simulink model "EMT"  (R2024b)
settings: Solver=ode5  StartTime=0.0  StopTime=1500  FixedStep=0.002  RelTol=1e-3
PreLoadFcn:
  | parameter;
InitFcn:
  | parameter;
StopFcn:
  | save('result.mat');
values from neighbouring files (symbols this model uses):
  A = 7.3    [parameter.m]
  a11 = (1+k1)*(1+k2)/k1/k2/iq    (= 1.54241568346)    [parameter.m]
  a11_L = a11    (= 1.54241568346)    [parameter.m]
  a12 = -(1+k1+k2)*(1+k3)/k1/k2    (= -3.86074191629)    [parameter.m]
  a12_L = a11*(1+k3+k4)/(1+k3)    (= 2.43173643789)    [parameter.m]
  a21 = -(1+k2)/k1/iq    (= -1.04963112005)    [parameter.m]
  a22 = (1+k1+k2)/k1    (= 2.46948356808)    [parameter.m]
  B = 2.71    [parameter.m]
  b11 = 0    [parameter.m]
  b12 = (1+k3)    (= 3.33)    [parameter.m]
  b21 = (1+k2)/iq    (= 2.23571428571)    [parameter.m]
  b22 = -k2    (= -2.13)    [parameter.m]
  C1_shift = 200    [parameter.m]
  Cb = 70    [parameter.m]
  Cd = 0.6    [parameter.m]
  eff_generator = eff_motor    [parameter.m]
  eff_motor = [0.80 0.80 0.84 0.84 0.83 0.85 0.83 0.83 0.83 0.80 0.80 0.80 ... (first row only)    [parameter.m]
  ele_map = [10.00,11.46,14.13,19.24,20.94,23.21,20.29,20.23,22.28,17.66,16.24,18.95,20.79,16.98,18.22,16.52,18.29,20.67,20.82,23.14,23.36,21.30,17.71,20.26,19.53,21.18,23.13,22.79,19.35,16.77,20.50,19.02,20.56,21.90,23.91,20.40,18.45,22.70,22.38,22.48,21.84,17.76,20.13,22.61,19.35,19.36,21.56,20.37,18.38,17.96,18.38,17.24,18.99,22.31,23.50,18.24,22.11,20.73,20.35,18.91,22.88,20.92,18.75,16.85,21.94,17.80,19. ...(+2007 chars)    [parameter.m]
  Fb_max = 5.5*mass    (= 247500)    [parameter.m]
  ic = 4.42    [parameter.m]
  JA = 0.4    [parameter.m]
  JB = JA    (= 0.4)    [parameter.m]
  Jc3r4 = 1e-2    (= 0.01)    [parameter.m]
  Je = 2.5    [parameter.m]
  Jh = 1e-2    (= 0.01)    [parameter.m]
  kh = 2.88    [parameter.m]
  kt = 1.83    [parameter.m]
  L = 4.472    [parameter.m]
  mass = 45000    [parameter.m]
  miu_max = 0.8    [parameter.m]
  n_generator = n_motor    [parameter.m]
  n_motor = [0 0.1 0.25 0.4 0.55 0.7 0.85 1 1.15 1.3 1.45 2.2]*3185    [parameter.m]
  nA_map = [-6000:50:-3250 -3200 0 3200 3250:50:6000]    [parameter.m]    (also in plot_result.m = [-7000:50:-3250 -3200 0 3200 3250:50:7000])
  nA_max = max(nA_map)    [parameter.m]
  nA_min = min(nA_map)    [parameter.m]
  nB_map = nA_map    [parameter.m]    (also in plot_result.m = [-7000:50:-3250 -3200 0 3200 3250:50:7000])
  nB_max = nA_max    [parameter.m]
  nB_min = nA_min    [parameter.m]
  ne_idl = 3000    [parameter.m]
  ne_map = [1600,1700,1800,1900,2000,2100,2200,2300,2400,2500,2600,2700,2800,2900,3000,3100,3200,3300,3400,3500,3600,3700,3800,3900,4000,4100,4200,4500]    [parameter.m]
  ne_max = 4200    [parameter.m]
  ne_min = 1600    [parameter.m]
  ne_start = 200    [parameter.m]
  nZ_map = [-8000:50:-4850 -4800 0 4800 4850:50:8000]    [parameter.m]
  Pb_epr = [-45 -45 -40 -30 0 30 40 45 45]    [parameter.m]
  Pb_max = [0 40 45 45 45]    [parameter.m]
  Pb_min = [-45 -45 -45 -40 0]    [parameter.m]
  Pe_ass = 210+20    (= 230)    [parameter.m]
  Pe_max = 1103    [parameter.m]
  PN0 = 0    [parameter.m]
  R_map = [0.90 0.89 0.90 0.91 0.92 0.93 0.94 0.95 0.96 0.97 0.98]/10    [parameter.m]
  rz = 0.318    [parameter.m]
  SOC0 = 60    [parameter.m]
  SOC_epr = [30 31 50 59 60 61 70 79 80]    [parameter.m]
  SOC_map = 0:10:100    [parameter.m]
  T_generator = T_motor    [parameter.m]
  T_motor = [0 0.3 0.8 1.3 1.8 2.3 2.8]/1.8*1110    [parameter.m]
  TA_max_map = [370*9549./(6000:-50:3250) 1110 1110 1110 370*9549./(3250:50:6000)]    [parameter.m]    (also in plot_result.m = [370*9549./(7000:-50:3250) 1100 1100 1100 370*9549./(3250:50)
  TA_min_map = -TA_max_map    [parameter.m]
  TAf = 0    [parameter.m]
  TB_max_map = TA_max_map    [parameter.m]    (also in plot_result.m = [370*9549./(7000:-50:3250) 1110 1110 1110 370*9549./(3250:50)
  TB_min_map = TA_min_map    [parameter.m]
  TBf = TAf    (= 0)    [parameter.m]
  Te_map = [0,599,798,998,1168,1324,1495,1660,1822,1970,2106,2235,2355,2458,2508,2543,2565,2606,2613,2649,2658,2689,2701,2707,2719,2724,2728,2740,2743,2754]    [parameter.m]
  Te_max_map = [1168,1324,1495,1660,1822,1970,2106,2235,2355,2458,2543,2606,2658,2701,2728,2743,2754,2743,2740,2724,2719,2707,2689,2649,2613,2565,2508,998]    [parameter.m]
  Te_start = 1600    [parameter.m]
  Tef = 100    [parameter.m]
  Time = 0:0.1:200    [parameter.m]
  Time_ele = 0:4:1600    [parameter.m]
  TS_A = 0.2    [parameter.m]
  TS_B = TS_A    (= 0.2)    [parameter.m]
  TS_C0 = 0.2    [parameter.m]
  TS_C1 = 0.2    [parameter.m]
  Ts_e = 0.1    [parameter.m]
  TS_Z1 = 0.2    [parameter.m]
  TS_Z2 = 0.2    [parameter.m]
  TZ_max_map = [450*9549./(8000:-50:4850) 1000 1000 1000 450*9549./(4850:50:8000)]    [parameter.m]
  TZ_min_map = -TZ_max_map    [parameter.m]
  Uoc_map = [3.258,3.668,3.733,3.783,3.833,3.877,3.912,3.941,3.973,4.013,4.200]*250    [parameter.m]
  v_cyc = 0.*(0<=Time&Time<11)+(3.75.*Time-41.25).*(11<=Time&Time<15)+15.*(15<=Time&Time<23)+(-3.*Time+84).*(23<=Time&Time<28)+0.*(28<=Time&Time<49)+(8.*Time/3-392/3).*(49<=Time&Time<61)+32.*(61<=Time&Time<85)+(-32.*Time/11+3072/11).*(85<=Time&Time<96)+0.*(96<=Time&Time<117)+(25.*Time/13-2925/13).*(117<=Time&Time<143)+50.*(143<=Time&Time<155)+(-15.*Time/8+2725/8).*(155<=Time&Time<163)+35.*(163<=Time&Time<17 ...(+70 chars)    [parameter.m]
  V_Shift12 = 32    [parameter.m]
  V_Shift21 = 25    [parameter.m]
  Voltage_epr = [750 760 900 1000 1050]    [parameter.m]
  Y_engine = 0.955    [parameter.m]
  Yc = 0.98    [parameter.m]
  Yh = 0.96    [parameter.m]
  Z1_shift = 200    [parameter.m]
  Z2_shift = 200    [parameter.m]
undefined symbols (not defined in the file or in its folder): sigbuilder_block
libraries: fl_lib x82, nesl_utility x55, simulink x49, sdl_lib x10, simulink_need_slupdate x6, powerlib_extras x1
(part 4 of 6)

== system EMT/Vehicle dynamics/vehicle dynamic/vehicle dynamic/Torque Actuator ==
  torque : Inport
  Ideal Torque Source : fl_lib/Mechanical/Mechanical Sources/Ideal Torque Source
  Mechanical Rotational Reference : fl_lib/Mechanical/Rotational Elements/Mechanical Rotational Reference
  Simulink-PS Converter : nesl_utility/Simulink-PS Converter  PhysicalDomain=network_engine_domain  SubClassName=ps_input  LeftPortType=input  RightPortType=output  PseudoPeriodic=off  Frequencies=[]  NoiseDistribution=none  NoiseParameters=[]  Unit=1  AffineConversion=off  FilteringAndDerivatives=filter  SimscapeFilterOrder=2  InputFilterTimeConstant=.001  UdotUserProvided=1
  shaft : PMIOPort  Side=Right
  wires:
  torque/1 -> Simulink-PS Converter/1
  connections:
  Simulink-PS Converter/RConn1 -- Ideal Torque Source/RConn1
  Mechanical Rotational Reference/LConn1 -- Ideal Torque Source/RConn2
  shaft/RConn1 -- Ideal Torque Source/LConn1

== system EMT/Vehicle dynamics/vehicle dynamic/vehicle dynamic/Torque Sensor ==
  Ideal Torque Sensor : fl_lib/Mechanical/Mechanical Sensors/Ideal Torque Sensor
  PS-Simulink Converter : nesl_utility/PS-Simulink Converter  PhysicalDomain=network_engine_domain  SubClassName=ps_output  LeftPortType=input  RightPortType=output  PseudoPeriodic=off  Frequencies=[]  VectorFormat=1-D array  Unit=1  AffineConversion=off
  In : PMIOPort  Side=Left
  Out : PMIOPort  Port=2  Side=Right
  Nm : Outport
  wires:
  PS-Simulink Converter/1 -> Nm/1
  connections:
  PS-Simulink Converter/LConn1 -- Ideal Torque Sensor/RConn2
  In/RConn1 -- Ideal Torque Sensor/LConn1
  Ideal Torque Sensor/RConn1 -- Out/RConn1

== system EMT/Vehicle dynamics/vehicle dynamic/vehicle dynamic/Wind Resistance ==
  Air Resistance : Fcn  Expr=0.5*Cd*A*u*u/21.15
  Memory3 : Memory
  Fw : Outport
  wires:
  [v_act] -> Memory3/1
  Memory3/1 -> Air Resistance/1
  Air Resistance/1 -> Fw/1

== system EMT/Vehicle dynamics/vehicle dynamic/vehicle dynamic1/Grade Resistance ==
  angle : Inport
  Ground Resistance : Fcn  Expr=0.5*mass*9.8*sin(u)
  Fg : Outport
  wires:
  angle/1 -> Ground Resistance/1
  Ground Resistance/1 -> Fg/1

== system EMT/Vehicle dynamics/vehicle dynamic/vehicle dynamic1/Ground Resistance ==
  fg : Inport
  angle : Inport  Port=2
  Ground Resistance : Fcn  Expr=0.5*u(1)*mass*9.8*cos(u(2))
  Mux : Mux  Inputs=2
  Ff : Outport
  wires:
  angle/1 -> Mux/2
  fg/1 -> Mux/1
  Mux/1 -> Ground Resistance/1
  Ground Resistance/1 -> Ff/1

== system EMT/Vehicle dynamics/vehicle dynamic/vehicle dynamic1/Mode Judge ==
  v : Inport
  Add : Sum  Inputs=+++
  Compare To Constant1 : simulink/Logic and Bit Operations/Compare To Constant  relop=<  const=-0.1  OutDataTypeStr=uint8
  Compare To Constant2 : simulink/Logic and Bit Operations/Compare To Constant  relop=>  const=0.1  OutDataTypeStr=uint8
  Compare To Constant3 : simulink/Logic and Bit Operations/Compare To Constant  relop=>=  const=-0.1  OutDataTypeStr=uint8
  Compare To Constant4 : simulink/Logic and Bit Operations/Compare To Constant  relop=<=  const=0.1  OutDataTypeStr=uint8
  Data Type Conversion : DataTypeConversion  SaturateOnIntegerOverflow=off  RndMeth=Floor
  Gain : Gain  Gain=3
  Gain1 : Gain  Gain=2
  Gain2 : Gain
  Logical Operator : Logic  AllPortsSameDT=off  OutDataTypeStr=boolean
  F : Outport
  wires:
  Gain2/1 -> Add/1
  Gain/1 -> Add/3
  Data Type Conversion/1 -> F/1
  Logical Operator/1 -> Gain/1
  Compare To Constant2/1 -> Gain1/1
  Compare To Constant4/1 -> Logical Operator/2
  Compare To Constant3/1 -> Logical Operator/1
  Compare To Constant1/1 -> Gain2/1
  v/1 -> Compare To Constant1/1, Compare To Constant2/1, Compare To Constant3/1, Compare To Constant4/1
  Add/1 -> Data Type Conversion/1
  Gain1/1 -> Add/2

== system EMT/Vehicle dynamics/vehicle dynamic/vehicle dynamic1/Speed Sensor ==
  Ideal Rotational Motion Sensor : fl_lib/Mechanical/Mechanical Sensors/Ideal Rotational Motion Sensor  reference=foundation.enum.MeasurementReference.difference  acceleration_port=false  velocity_port=true  position_port=true  wrap_angle=false  offset=0 rad
  PS-Simulink Converter : nesl_utility/PS-Simulink Converter  PhysicalDomain=network_engine_domain  SubClassName=ps_output  LeftPortType=input  RightPortType=output  PseudoPeriodic=off  Frequencies=[]  VectorFormat=1-D array  Unit=1  AffineConversion=off
  Reference : fl_lib/Mechanical/Rotational Elements/Mechanical Rotational Reference
  Tire Radius2 : Gain  Gain=30/pi
  shaft : PMIOPort  Side=Left
  r/min : Outport
  wires:
  PS-Simulink Converter/1 -> Tire Radius2/1
  Tire Radius2/1 -> r/min/1
  connections:
  PS-Simulink Converter/LConn1 -- Ideal Rotational Motion Sensor/RConn2
  Reference/LConn1 -- Ideal Rotational Motion Sensor/RConn1
  shaft/RConn1 -- Ideal Rotational Motion Sensor/LConn1

== system EMT/Vehicle dynamics/vehicle dynamic/vehicle dynamic1/Steering Resistance ==
  Abs : Abs  SaturateOnIntegerOverflow=off
  Compare To Constant : simulink/Logic and Bit Operations/Compare To Constant  relop=>=  const=10^3  OutDataTypeStr=uint8  ZeroCross=off
  Constant1 : Constant  Value=0
  Memory1 : Memory
  Memory3 : Memory
  Mux : Mux  Inputs=2
  Product2 : Product  RndMeth=Zero
  Sign1 : Signum
  Steering Resistance : Fcn  Expr=miu_max/(0.925+0.15*(u))*mass*9.8*L/4/B
  Switch : Switch  Threshold=0.5  SaturateOnIntegerOverflow=off  InputSameDT=off
  rou : Fcn  Expr=(u(1)+u(2))/(u(2)-u(1)+0.1^10)/2
  Fs : Outport
  wires:
  [v_Right] -> Memory1/1
  [v_Left] -> Memory3/1
  Product2/1 -> Fs/1
  Sign1/1 -> Switch/3
  Switch/1 -> Product2/2
  Constant1/1 -> Switch/1
  Compare To Constant/1 -> Switch/2
  Abs/1 -> Steering Resistance/1  "rou"
  rou/1 -> Sign1/1, Compare To Constant/1, Abs/1
  Mux/1 -> rou/1
  Memory1/1 -> Mux/2
  Memory3/1 -> Mux/1
  Steering Resistance/1 -> Product2/1

== system EMT/Vehicle dynamics/vehicle dynamic/vehicle dynamic1/Torque Actuator ==
  torque : Inport
  Ideal Torque Source : fl_lib/Mechanical/Mechanical Sources/Ideal Torque Source
  Mechanical Rotational Reference : fl_lib/Mechanical/Rotational Elements/Mechanical Rotational Reference
  Simulink-PS Converter : nesl_utility/Simulink-PS Converter  PhysicalDomain=network_engine_domain  SubClassName=ps_input  LeftPortType=input  RightPortType=output  PseudoPeriodic=off  Frequencies=[]  NoiseDistribution=none  NoiseParameters=[]  Unit=1  AffineConversion=off  FilteringAndDerivatives=filter  SimscapeFilterOrder=2  InputFilterTimeConstant=.001  UdotUserProvided=1
  shaft : PMIOPort  Side=Right
  wires:
  torque/1 -> Simulink-PS Converter/1
  connections:
  shaft/RConn1 -- Ideal Torque Source/LConn1
  Mechanical Rotational Reference/LConn1 -- Ideal Torque Source/RConn2
  Simulink-PS Converter/RConn1 -- Ideal Torque Source/RConn1

== system EMT/Vehicle dynamics/vehicle dynamic/vehicle dynamic1/Torque Sensor ==
  Ideal Torque Sensor : fl_lib/Mechanical/Mechanical Sensors/Ideal Torque Sensor
  PS-Simulink Converter : nesl_utility/PS-Simulink Converter  PhysicalDomain=network_engine_domain  SubClassName=ps_output  LeftPortType=input  RightPortType=output  PseudoPeriodic=off  Frequencies=[]  VectorFormat=1-D array  Unit=1  AffineConversion=off
  In : PMIOPort  Side=Left
  Out : PMIOPort  Port=2  Side=Right
  Nm : Outport
  wires:
  PS-Simulink Converter/1 -> Nm/1
  connections:
  Ideal Torque Sensor/RConn1 -- Out/RConn1
  In/RConn1 -- Ideal Torque Sensor/LConn1
  PS-Simulink Converter/LConn1 -- Ideal Torque Sensor/RConn2

== system EMT/Vehicle dynamics/vehicle dynamic/vehicle dynamic1/Wind Resistance ==
  Air Resistance : Fcn  Expr=0.5*Cd*A*u*u/21.15
  Memory3 : Memory
  Fw : Outport
  wires:
  [v_act] -> Memory3/1
  Memory3/1 -> Air Resistance/1
  Air Resistance/1 -> Fw/1

== system EMT/engine/Engine/Subsystem1/Torque Actuator ==
  torque : Inport
  Ideal Torque Source : fl_lib/Mechanical/Mechanical Sources/Ideal Torque Source
  Mechanical Rotational Reference : fl_lib/Mechanical/Rotational Elements/Mechanical Rotational Reference
  Simulink-PS Converter : nesl_utility/Simulink-PS Converter  PhysicalDomain=network_engine_domain  SubClassName=ps_input  LeftPortType=input  RightPortType=output  PseudoPeriodic=off  Frequencies=[]  NoiseDistribution=none  NoiseParameters=[]  Unit=N*m  AffineConversion=off  FilteringAndDerivatives=zero  SimscapeFilterOrder=1  InputFilterTimeConstant=.001  UdotUserProvided=0
  shaft : PMIOPort  Side=Right
  wires:
  torque/1 -> Simulink-PS Converter/1
  connections:
  Simulink-PS Converter/RConn1 -- Ideal Torque Source/RConn1
  Mechanical Rotational Reference/LConn1 -- Ideal Torque Source/RConn2
  shaft/RConn1 -- Ideal Torque Source/LConn1

== system EMT/motorA/Motor/Mechanical Body/Max & Min Torque Control ==
  speed : Inport
  Tm_com : Inport  Port=2
  Lookup Table : Lookup  InputValues=nm_map  Table=Tm_max_map  SaturateOnIntegerOverflow=off
  Lookup Table1 : Lookup  InputValues=nm_map  Table=Tm_min_map  SaturateOnIntegerOverflow=off
  Saturation Dynamic : simulink/Discontinuities/Saturation Dynamic  OutMin=[]  OutMax=[]  OutDataTypeStr=Inherit: Same as second input  OutDataType=sfix(16)  OutScaling=2^-10  DoSatur=off
  Saturation1 : Saturate  UpperLimit=max(nm_map)  LowerLimit=min(nm_map)
  Saturation2 : Saturate  UpperLimit=max(nm_map)  LowerLimit=min(nm_map)
  Transfer Fcn : TransferFcn  Denominator=[T 1]
  torque : Outport
  wires:
  speed/1 -> Saturation2/1, Saturation1/1
  Lookup Table/1 -> Saturation Dynamic/1
  Lookup Table1/1 -> Saturation Dynamic/3
  Saturation1/1 -> Lookup Table/1
  Saturation2/1 -> Lookup Table1/1
  Tm_com/1 -> Saturation Dynamic/2
  Saturation Dynamic/1 -> Transfer Fcn/1
  Transfer Fcn/1 -> torque/1

== system EMT/motorA/Motor/Mechanical Body/Resistance ==
  speed : Inport
  Constant2 : Constant  Value=-Tmf
  Product2 : Product  RndMeth=Zero
  Sign2 : Signum
  Torque Actuator : Subsystem  mask(Torque Actuator){}
      mask help: The torque unit is Nm.
  Tmf : PMIOPort  Side=Right
  wires:
  speed/1 -> Sign2/1
  Product2/1 -> Torque Actuator/1(torque)
  Sign2/1 -> Product2/1
  Constant2/1 -> Product2/2
  connections:
  Tmf/RConn1 -- Torque Actuator/RConn1

== system EMT/motorA/Motor/Mechanical Body/Speed Sensor ==
  Ideal Rotational Motion Sensor : fl_lib/Mechanical/Mechanical Sensors/Ideal Rotational Motion Sensor  reference=foundation.enum.MeasurementReference.difference  acceleration_port=false  velocity_port=true  position_port=true  wrap_angle=false  offset=0 rad
  PS-Simulink Converter : nesl_utility/PS-Simulink Converter  PhysicalDomain=network_engine_domain  SubClassName=ps_output  LeftPortType=input  RightPortType=output  PseudoPeriodic=off  Frequencies=[]  VectorFormat=1-D array  Unit=rad/s  AffineConversion=off
  Reference : fl_lib/Mechanical/Rotational Elements/Mechanical Rotational Reference
  Tire Radius2 : Gain  Gain=30/pi
  shaft : PMIOPort  Side=Left
  r/min : Outport
  wires:
  Tire Radius2/1 -> r/min/1
  PS-Simulink Converter/1 -> Tire Radius2/1
  connections:
  shaft/RConn1 -- Ideal Rotational Motion Sensor/LConn1
  Reference/LConn1 -- Ideal Rotational Motion Sensor/RConn1
  PS-Simulink Converter/LConn1 -- Ideal Rotational Motion Sensor/RConn2

== system EMT/motorA/Motor/Mechanical Body/Torque Actuator ==
  torque : Inport
  Ideal Torque Source : fl_lib/Mechanical/Mechanical Sources/Ideal Torque Source
  Mechanical Rotational Reference : fl_lib/Mechanical/Rotational Elements/Mechanical Rotational Reference
  Simulink-PS Converter : nesl_utility/Simulink-PS Converter  PhysicalDomain=network_engine_domain  SubClassName=ps_input  LeftPortType=input  RightPortType=output  PseudoPeriodic=off  Frequencies=[]  NoiseDistribution=none  NoiseParameters=[]  Unit=N*m  AffineConversion=off  FilteringAndDerivatives=filter  SimscapeFilterOrder=1  InputFilterTimeConstant=.001  UdotUserProvided=1
  shaft : PMIOPort  Side=Right
  wires:
  torque/1 -> Simulink-PS Converter/1
  connections:
  shaft/RConn1 -- Ideal Torque Source/LConn1
  Mechanical Rotational Reference/LConn1 -- Ideal Torque Source/RConn2
  Simulink-PS Converter/RConn1 -- Ideal Torque Source/RConn1

== system EMT/motorB/Motor/Mechanical Body/Max & Min Speed Control ==
  speed : Inport
  Tm_com : Inport  Port=2
  Lookup Table : Lookup  InputValues=nm_map  Table=Tm_max_map  SaturateOnIntegerOverflow=off
  Lookup Table1 : Lookup  InputValues=nm_map  Table=Tm_min_map  SaturateOnIntegerOverflow=off
  Saturation Dynamic : simulink/Discontinuities/Saturation Dynamic  OutMin=[]  OutMax=[]  OutDataTypeStr=Inherit: Same as second input  OutDataType=sfix(16)  OutScaling=2^-10  DoSatur=off
  Saturation1 : Saturate  UpperLimit=max(nm_map)  LowerLimit=min(nm_map)
  Saturation2 : Saturate  UpperLimit=max(nm_map)  LowerLimit=min(nm_map)
  Transfer Fcn : TransferFcn  Denominator=[T 1]
  torque : Outport
  wires:
  Transfer Fcn/1 -> torque/1
  speed/1 -> Saturation2/1, Saturation1/1
  Lookup Table/1 -> Saturation Dynamic/1
  Lookup Table1/1 -> Saturation Dynamic/3
  Saturation1/1 -> Lookup Table/1
  Saturation2/1 -> Lookup Table1/1
  Tm_com/1 -> Saturation Dynamic/2
  Saturation Dynamic/1 -> Transfer Fcn/1

== system EMT/motorB/Motor/Mechanical Body/Resistance ==
  speed : Inport
  Constant2 : Constant  Value=-Tmf
  Product2 : Product  RndMeth=Zero
  Sign2 : Signum
  Torque Actuator : Subsystem  mask(Torque Actuator){}
      mask help: The torque unit is Nm.
  Tmf : PMIOPort  Side=Right
  wires:
  speed/1 -> Sign2/1
  Product2/1 -> Torque Actuator/1(torque)
  Sign2/1 -> Product2/1
  Constant2/1 -> Product2/2
  connections:
  Tmf/RConn1 -- Torque Actuator/RConn1

== system EMT/motorB/Motor/Mechanical Body/Speed Sensor ==
  Ideal Rotational Motion Sensor : fl_lib/Mechanical/Mechanical Sensors/Ideal Rotational Motion Sensor  reference=foundation.enum.MeasurementReference.difference  acceleration_port=false  velocity_port=true  position_port=true  wrap_angle=false  offset=0 rad
  PS-Simulink Converter : nesl_utility/PS-Simulink Converter  PhysicalDomain=network_engine_domain  SubClassName=ps_output  LeftPortType=input  RightPortType=output  PseudoPeriodic=off  Frequencies=[]  VectorFormat=1-D array  Unit=rad/s  AffineConversion=off
  Reference : fl_lib/Mechanical/Rotational Elements/Mechanical Rotational Reference
  Tire Radius2 : Gain  Gain=30/pi
  shaft : PMIOPort  Side=Left
  r/min : Outport
  wires:
  Tire Radius2/1 -> r/min/1
  PS-Simulink Converter/1 -> Tire Radius2/1
  connections:
  shaft/RConn1 -- Ideal Rotational Motion Sensor/LConn1
  Reference/LConn1 -- Ideal Rotational Motion Sensor/RConn1
  PS-Simulink Converter/LConn1 -- Ideal Rotational Motion Sensor/RConn2

== system EMT/motorB/Motor/Mechanical Body/Torque Actuator ==
  torque : Inport
  Ideal Torque Source : fl_lib/Mechanical/Mechanical Sources/Ideal Torque Source
  Mechanical Rotational Reference : fl_lib/Mechanical/Rotational Elements/Mechanical Rotational Reference
  Simulink-PS Converter : nesl_utility/Simulink-PS Converter  PhysicalDomain=network_engine_domain  SubClassName=ps_input  LeftPortType=input  RightPortType=output  PseudoPeriodic=off  Frequencies=[]  NoiseDistribution=none  NoiseParameters=[]  Unit=N*m  AffineConversion=off  FilteringAndDerivatives=filter  SimscapeFilterOrder=1  InputFilterTimeConstant=.001  UdotUserProvided=1
  shaft : PMIOPort  Side=Right
  wires:
  torque/1 -> Simulink-PS Converter/1
  connections:
  shaft/RConn1 -- Ideal Torque Source/LConn1
  Mechanical Rotational Reference/LConn1 -- Ideal Torque Source/RConn2
  Simulink-PS Converter/RConn1 -- Ideal Torque Source/RConn1

== system EMT/Control Unit/Control/EVT1_H Stage/clutches condition/Subsystem ==
  Constant1 : Constant
  C0 : Outport
  wires:
  Constant1/1 -> C0/1

== system EMT/Control Unit/Control/EVT1_H Stage/clutches condition/Subsystem1 ==
  Constant1 : Constant
  Z2 : Outport
  wires:
  Constant1/1 -> Z2/1

== system EMT/Control Unit/Control/EVT1_H Stage/clutches condition/Subsystem2 ==
  Compare To Constant1 : simulink/Logic and Bit Operations/Compare To Constant  relop=<  const=C1_shift  OutDataTypeStr=uint8
  Data Type Conversion : DataTypeConversion  SaturateOnIntegerOverflow=off  RndMeth=Floor
  Fcn : Fcn  Expr=V_Shift12+5*(u-1)
  Logical Operator1 : Logic  AllPortsSameDT=off  OutDataTypeStr=boolean
  Memory1 : Memory
  Memory2 : Memory
  Memory5 : Memory
  Relational Operator : RelationalOperator  OutDataTypeStr=boolean  InputSameDT=off
  C1 : Outport
  wires:
  Logical Operator1/1 -> Data Type Conversion/1
  Compare To Constant1/1 -> Logical Operator1/2
  Relational Operator/1 -> Logical Operator1/1
  Fcn/1 -> Relational Operator/2
  Memory1/1 -> Fcn/1
  [Acc_pedal] -> Memory1/1
  Memory2/1 -> Relational Operator/1
  Memory5/1 -> Compare To Constant1/1
  [C1_rela] -> Memory5/1
  Data Type Conversion/1 -> C1/1
  [v_act] -> Memory2/1

== system EMT/Control Unit/Control/EVT1_H Stage/clutches condition/Subsystem4 ==
  Constant1 : Constant  Value=0
  Z1 : Outport
  wires:
  Constant1/1 -> Z1/1

== system EMT/Control Unit/Control/EVT1_H Stage/engine torque/Subsystem1 ==
  Te_ref : Inport
  ne_act : Inport  Port=2
  Constant : Constant  Value=ne_idl
  Constant1 : Constant  Value=0
  Lookup Table : Lookup  InputValues=ne_map  Table=Te_max_map  SaturateOnIntegerOverflow=off
  Memory1 : Memory
  Memory5 : Memory
  PID Controller2 : simulink_need_slupdate/PID Controller  P=4  I=0.01  D=10
  Saturation : Saturate  UpperLimit=max(ne_map)  LowerLimit=min(ne_map)
  Saturation Dynamic : simulink/Discontinuities/Saturation Dynamic  OutMin=[]  OutMax=[]  OutDataTypeStr=Inherit: Same as second input  OutDataType=sfix(16)  OutScaling=2^-10  DoSatur=off
  Sum1 : Sum  Inputs=+-
  Switch : Switch  Criteria=u2 > Threshold  Threshold=10  SaturateOnIntegerOverflow=off  InputSameDT=off
  ne_act1 : InportShadow  Port=2
  Te_com : Outport
  wires:
  Memory1/1 -> Saturation/1
  ne_act1/1 -> Memory1/1
  Switch/1 -> Saturation Dynamic/2
  Saturation Dynamic/1 -> Te_com/1
  Constant1/1 -> Saturation Dynamic/3
  Lookup Table/1 -> Saturation Dynamic/1
  Saturation/1 -> Lookup Table/1
  Constant/1 -> Sum1/1
  PID Controller2/1 -> Switch/3
  Te_ref/1 -> Switch/2, Switch/1
  Sum1/1 -> PID Controller2/1
  ne_act/1 -> Memory5/1
  Memory5/1 -> Sum1/2

== system EMT/Control Unit/Control/EVT2 Stage/clutches condition/Subsystem ==
  Constant1 : Constant
  C0 : Outport
  wires:
  Constant1/1 -> C0/1

== system EMT/Control Unit/Control/EVT2 Stage/clutches condition/Subsystem1 ==
  Compare To Constant1 : simulink/Logic and Bit Operations/Compare To Constant  relop=<  const=Z2_shift  OutDataTypeStr=uint8
  Data Type Conversion1 : DataTypeConversion  SaturateOnIntegerOverflow=off  RndMeth=Floor
  Fcn : Fcn  Expr=V_Shift21+5*u
  Logical Operator1 : Logic  AllPortsSameDT=off  OutDataTypeStr=boolean
  Memory1 : Memory
  Memory2 : Memory
  Memory5 : Memory
  Relational Operator : RelationalOperator  Operator=<=  OutDataTypeStr=boolean  InputSameDT=off
  Z2 : Outport
  wires:
  Fcn/1 -> Relational Operator/2
  Memory1/1 -> Fcn/1
  [Acc_pedal] -> Memory1/1
  Data Type Conversion1/1 -> Z2/1
  Logical Operator1/1 -> Data Type Conversion1/1
  Compare To Constant1/1 -> Logical Operator1/2
  Relational Operator/1 -> Logical Operator1/1
  [v_act] -> Memory2/1
  Memory2/1 -> Relational Operator/1
  [Z2_rela] -> Memory5/1
  Memory5/1 -> Compare To Constant1/1

== system EMT/Control Unit/Control/EVT2 Stage/clutches condition/Subsystem2 ==
  Constant1 : Constant
  C1 : Outport
  wires:
  Constant1/1 -> C1/1

== system EMT/Control Unit/Control/EVT2 Stage/clutches condition/Subsystem4 ==
  Constant1 : Constant  Value=0
  Z1 : Outport
  wires:
  Constant1/1 -> Z1/1

== system EMT/Control Unit/Control/EVT2 Stage/motorZ torque/Subsystem1 ==
  nZ_act : Inport
  Constant3 : Constant  Value=0
  Memory5 : Memory
  PID Controller2 : simulink_need_slupdate/PID Controller  P=2  I=0.01  D=0.1
  Sum1 : Sum  Inputs=+-
  TZ_com : Outport
  wires:
  Memory5/1 -> Sum1/2
  Constant3/1 -> Sum1/1
  nZ_act/1 -> Memory5/1
  Sum1/1 -> PID Controller2/1
  PID Controller2/1 -> TZ_com/1

== system EMT/Control Unit/Control/Power Distribution/Electric Power Requirement/Data ==
  PN_com : Inport
  PN_max : Inport  Port=2
  PN_min : Inport  Port=3
  tag scope: PN_com=global, PN_max=global, PN_min=global
  wires:
  PN_min/1 -> [PN_min]
  PN_max/1 -> [PN_max]
  PN_com/1 -> [PN_com]

== system EMT/Control Unit/Control/Power Distribution/Feasible Control Range/State Calculation ==
  s : Inport
  ne : Inport  Port=2
  v_act : Inport  Port=3
  Speed : Subsystem
  Subsystem3 : Subsystem
  no1 : Fcn  Expr=u*(1+kh)/kh*ic/0.377/rz
  stage : Outport
  ne_act : Outport  Port=2
  nA_act : Outport  Port=3
  nB_act : Outport  Port=4
  no_act : Outport  Port=5
  wires:
  Speed/2(nB) -> nB_act/1
  Speed/1(nA) -> nA_act/1
  ne/1 -> ne_act/1, Speed/2(ne)
  no1/1 -> no_act/1, Speed/3(no)
  Subsystem3/1(1) -> Speed/1(stage)
  s/1 -> stage/1, Subsystem3/1(0)
  v_act/1 -> no1/1

== system EMT/Control Unit/Control/Power Distribution/Feasible Control Range/State Predition ==
  stage : Inport
  ne_act : Inport  Port=2
  nA_act : Inport  Port=3
  nB_act : Inport  Port=4
  no_act : Inport  Port=5
  TA Range : Subsystem
  TB Range : Subsystem
  Te Range : Subsystem
  Z : Subsystem
  ne_act2 : InportShadow  Port=2
  stage_k : Outport
  ne_k : Outport  Port=2
  no_k : Outport  Port=3
  Te_k : Outport  Port=4
  TA_k : Outport  Port=5
  TB_k : Outport  Port=6
  wires:
  ne_act/1 -> Te Range/1(ne_act)
  Te Range/1(Te_k) -> Te_k/1
  nA_act/1 -> TA Range/1(nA)
  TA Range/1(TA_R) -> TA_k/1
  nB_act/1 -> TB Range/1(nB)
  TB Range/1(TB_R) -> TB_k/1
  Z/1(ne_k) -> ne_k/1
  stage/1 -> Z/1(stage), stage_k/1
  ne_act2/1 -> Z/2(ne_act)
  no_act/1 -> Z/3(no_act), no_k/1

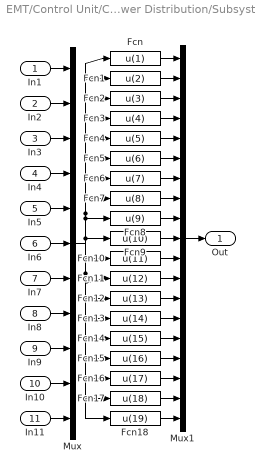
== system EMT/Control Unit/Control/Power Distribution/Optimal Power Distribution/Subsystem ==
  In1 : Inport
  In2 : Inport  Port=2
  In3 : Inport  Port=3
  In4 : Inport  Port=4
  In5 : Inport  Port=5
  In6 : Inport  Port=6
  In7 : Inport  Port=7
  In8 : Inport  Port=8
  In9 : Inport  Port=9
  In10 : Inport  Port=10
  In11 : Inport  Port=11
  Fcn : Fcn  Expr=u(1)
  Fcn1 : Fcn  Expr=u(2)
  Fcn10 : Fcn  Expr=u(11)
  Fcn11 : Fcn  Expr=u(12)
  Fcn12 : Fcn  Expr=u(13)
  Fcn13 : Fcn  Expr=u(14)
  Fcn14 : Fcn  Expr=u(15)
  Fcn15 : Fcn  Expr=u(16)
  Fcn16 : Fcn  Expr=u(17)
  Fcn17 : Fcn  Expr=u(18)
  Fcn18 : Fcn  Expr=u(19)
  Fcn2 : Fcn  Expr=u(3)
  Fcn3 : Fcn  Expr=u(4)
  Fcn4 : Fcn  Expr=u(5)
  Fcn5 : Fcn  Expr=u(6)
  Fcn6 : Fcn  Expr=u(7)
  Fcn7 : Fcn  Expr=u(8)
  Fcn8 : Fcn  Expr=u(9)
  Fcn9 : Fcn  Expr=u(10)
  Mux : Mux  Inputs=11
  Mux1 : Mux  Inputs=19
  Out : Outport
  wires:
  In9/1 -> Mux/9
  In8/1 -> Mux/8
  In7/1 -> Mux/7
  Mux1/1 -> Out/1
  In6/1 -> Mux/6
  In5/1 -> Mux/5
  In4/1 -> Mux/4
  In3/1 -> Mux/3
  In2/1 -> Mux/2
  In1/1 -> Mux/1
  Fcn15/1 -> Mux1/16
  Fcn14/1 -> Mux1/15
  Fcn13/1 -> Mux1/14
  Fcn12/1 -> Mux1/13
  Fcn11/1 -> Mux1/12
  Fcn10/1 -> Mux1/11
  Fcn9/1 -> Mux1/10
  Fcn8/1 -> Mux1/9
  Fcn7/1 -> Mux1/8
  Fcn6/1 -> Mux1/7
  Fcn5/1 -> Mux1/6
  Fcn4/1 -> Mux1/5
  Fcn3/1 -> Mux1/4
  Fcn2/1 -> Mux1/3
  Fcn1/1 -> Mux1/2
  Fcn/1 -> Mux1/1
  In10/1 -> Mux/10
  Fcn16/1 -> Mux1/17
  Fcn17/1 -> Mux1/18
  Mux/1 -> Fcn10/1, Fcn9/1, Fcn7/1, Fcn6/1, Fcn5/1, Fcn4/1, Fcn3/1, Fcn2/1, Fcn1/1, Fcn/1, Fcn14/1, Fcn15/1, Fcn16/1, Fcn17/1, Fcn18/1, Fcn13/1, Fcn12/1, Fcn11/1, Fcn8/1
  Fcn18/1 -> Mux1/19
  In11/1 -> Mux/11

== system EMT/Control Unit/Control/Power Distribution/Pedal Interpretation/Brake Control ==
  Dec_pedal : Inport
  Constant : Constant  Value=0
  Fcn1 : Fcn  Expr=Fb_max*u^2
  Switch : Switch  SaturateOnIntegerOverflow=off  InputSameDT=off
  Fb_ref : Outport
  wires:
  Dec_pedal/1 -> Switch/2, Fcn1/1
  Switch/1 -> Fb_ref/1
  Fcn1/1 -> Switch/3
  Constant/1 -> Switch/1

== system EMT/Control Unit/Control/Power Distribution/Pedal Interpretation/Data ==
  Dec_pedal : Inport
  Acc_pedal : Inport  Port=2
  Pe_com : Inport  Port=3
  tag scope: Acc_pedal=global, Dec_pedal=global, Pe_com=global
  wires:
  Acc_pedal/1 -> [Acc_pedal]
  Dec_pedal/1 -> [Dec_pedal]
  Pe_com/1 -> [Pe_com]

== system EMT/Control Unit/Control/Power Distribution/Pedal Interpretation/Engine Power Requirement ==
  Acc_pedal : Inport
  Constant : Constant  Value=0
  Fcn : Fcn  Expr=Pe_max*u^2
  Switch1 : Switch  SaturateOnIntegerOverflow=off  InputSameDT=off
  Pe_com : Outport
  wires:
  Constant/1 -> Switch1/3
  Fcn/1 -> Switch1/1
  Acc_pedal/1 -> Switch1/2, Fcn/1
  Switch1/1 -> Pe_com/1

== system EMT/Control Unit/Control/Power Distribution/Pedal Interpretation/Subsystem7 ==
  0 : Inport
  Constant : Constant  Value=0
  MinMax : MinMax  Function=max  Inputs=2
  1 : Outport
  wires:
  MinMax/1 -> 1/1
  0/1 -> MinMax/1
  Constant/1 -> MinMax/2

== system EMT/Control Unit/Control/Power Distribution/Pedal Interpretation/Subsystem8 ==
  0 : Inport
  Constant : Constant  Value=0
  MinMax : MinMax  Inputs=2
  1 : Outport
  wires:
  Constant/1 -> MinMax/2
  0/1 -> MinMax/1
  MinMax/1 -> 1/1

== system EMT/Control Unit/Control/Prepare Stage/clutches condition/Subsystem ==
  Constant1 : Constant
  C0 : Outport
  wires:
  Constant1/1 -> C0/1

== system EMT/Control Unit/Control/Prepare Stage/clutches condition/Subsystem1 ==
  Compare To Constant1 : simulink/Logic and Bit Operations/Compare To Constant  relop=<  const=0.5  OutDataTypeStr=uint8
  Compare To Constant2 : simulink/Logic and Bit Operations/Compare To Constant  relop=<=  const=0.5  OutDataTypeStr=boolean
  Compare To Constant3 : simulink/Logic and Bit Operations/Compare To Constant  relop=<  const=Z2_shift  OutDataTypeStr=boolean
  Compare To Constant4 : simulink/Logic and Bit Operations/Compare To Constant  relop=<  const=0.5  OutDataTypeStr=uint8
  Constant : Constant  Value=ne_idl
  Data Type Conversion : DataTypeConversion  SaturateOnIntegerOverflow=off  RndMeth=Floor
  Logical Operator1 : Logic  Inputs=5  AllPortsSameDT=off  OutDataTypeStr=boolean
  Memory3 : Memory
  Memory4 : Memory
  Relational Operator : RelationalOperator  OutDataTypeStr=boolean  InputSameDT=off
  Z2 : Outport
  wires:
  Compare To Constant1/1 -> Logical Operator1/5
  Compare To Constant4/1 -> Logical Operator1/4
  [Center_Steering] -> Compare To Constant1/1
  [Generating_Knob] -> Compare To Constant4/1
  Data Type Conversion/1 -> Z2/1
  Constant/1 -> Relational Operator/2
  Compare To Constant2/1 -> Logical Operator1/3
  [Z2_rela] -> Memory3/1
  Memory3/1 -> Compare To Constant3/1
  Compare To Constant3/1 -> Logical Operator1/2
  Logical Operator1/1 -> Data Type Conversion/1
  [ne_act] -> Memory4/1
  Relational Operator/1 -> Logical Operator1/1
  Memory4/1 -> Relational Operator/1
  [Grade_Gear] -> Compare To Constant2/1

== system EMT/Control Unit/Control/Prepare Stage/clutches condition/Subsystem2 ==
  Constant1 : Constant  Value=0
  C1 : Outport
  wires:
  Constant1/1 -> C1/1

== system EMT/Control Unit/Control/Prepare Stage/clutches condition/Subsystem3 ==
  Compare To Constant1 : simulink/Logic and Bit Operations/Compare To Constant  relop=<  const=0.5  OutDataTypeStr=uint8
  Compare To Constant2 : simulink/Logic and Bit Operations/Compare To Constant  relop=>  const=0.5  OutDataTypeStr=boolean
  Compare To Constant3 : simulink/Logic and Bit Operations/Compare To Constant  relop=<  const=Z1_shift  OutDataTypeStr=boolean
  Compare To Constant4 : simulink/Logic and Bit Operations/Compare To Constant  relop=<  const=0.5  OutDataTypeStr=uint8
  Constant : Constant  Value=ne_idl
  Data Type Conversion : DataTypeConversion  SaturateOnIntegerOverflow=off  RndMeth=Floor
  Logical Operator1 : Logic  Inputs=5  AllPortsSameDT=off  OutDataTypeStr=boolean
  Memory2 : Memory
  Memory3 : Memory
  Relational Operator1 : RelationalOperator  OutDataTypeStr=boolean  InputSameDT=off
  Z1 : Outport
  wires:
  Compare To Constant1/1 -> Logical Operator1/5
  Compare To Constant4/1 -> Logical Operator1/4
  [Center_Steering] -> Compare To Constant1/1
  [Generating_Knob] -> Compare To Constant4/1
  Relational Operator1/1 -> Logical Operator1/1
  Constant/1 -> Relational Operator1/2
  [ne_act] -> Memory2/1
  Memory2/1 -> Relational Operator1/1
  Data Type Conversion/1 -> Z1/1
  [Grade_Gear] -> Compare To Constant2/1
  Compare To Constant2/1 -> Logical Operator1/3
  Logical Operator1/1 -> Data Type Conversion/1
  Compare To Constant3/1 -> Logical Operator1/2
  Memory3/1 -> Compare To Constant3/1
  [Z1_rela] -> Memory3/1

== system EMT/Control Unit/Control/Prepare Stage/engine swich/Triggered Subsystem ==
  In1 : Inport
  Trigger : TriggerPort  VariantControl=Variant
  Out1 : Outport
  wires:
  In1/1 -> Out1/1

== system EMT/Control Unit/Control/Prepare Stage/engine torque/Subsystem1 ==
  ne_act : Inport
  Constant : Constant  Value=ne_idl
  Constant1 : Constant  Value=0
  Lookup Table : Lookup  InputValues=ne_map  Table=Te_max_map  SaturateOnIntegerOverflow=off
  Memory2 : Memory
  PID Controller2 : simulink_need_slupdate/PID Controller  P=4  I=0.01  D=10
  Saturation : Saturate  UpperLimit=max(ne_map)  LowerLimit=min(ne_map)
  Saturation Dynamic : simulink/Discontinuities/Saturation Dynamic  OutMin=[]  OutMax=[]  OutDataTypeStr=Inherit: Same as second input  OutDataType=sfix(16)  OutScaling=2^-10  DoSatur=off
  Sum1 : Sum  Inputs=-+
  Te_com : Outport
  wires:
  Memory2/1 -> Saturation/1, Sum1/1
  ne_act/1 -> Memory2/1
  Constant/1 -> Sum1/2
  PID Controller2/1 -> Saturation Dynamic/2
  Saturation Dynamic/1 -> Te_com/1
  Constant1/1 -> Saturation Dynamic/3
  Lookup Table/1 -> Saturation Dynamic/1
  Saturation/1 -> Lookup Table/1
  Sum1/1 -> PID Controller2/1

== system EMT/Control Unit/Control/Prepare Stage/motorA torque/Subsystem ==
  Compare To Constant1 : simulink/Logic and Bit Operations/Compare To Constant  relop=>=  const=0.9  OutDataTypeStr=uint8
  Data Type Conversion : DataTypeConversion  SaturateOnIntegerOverflow=off  RndMeth=Floor
  Memory2 : Memory
  Judge : Outport
  wires:
  Data Type Conversion/1 -> Judge/1
  [Press_C0] -> Memory2/1
  Memory2/1 -> Compare To Constant1/1
  Compare To Constant1/1 -> Data Type Conversion/1

== system EMT/Control Unit/Control/Prepare Stage/motorA torque/TA_com1 ==
  Lookup Table : Lookup  InputValues=nA_map  Table=TA_max_map*1.5  SaturateOnIntegerOverflow=off
  Lookup Table1 : Lookup  InputValues=nA_map  Table=TA_min_map*1.5  SaturateOnIntegerOverflow=off
  MinMax : MinMax  Inputs=2
  Saturation Dynamic : simulink/Discontinuities/Saturation Dynamic  OutMin=[]  OutMax=[]  OutDataTypeStr=Inherit: Same as second input  OutDataType=sfix(16)  OutScaling=2^-10  DoSatur=off
  Saturation1 : Saturate  UpperLimit=max(nA_map)  LowerLimit=min(nA_map)
  Saturation2 : Saturate  UpperLimit=max(nA_map)  LowerLimit=min(nA_map)
  Subsystem1 : Subsystem
  Subsystem2 : Subsystem
  TA_com : Outport
  wires:
  [PN_max] -> Subsystem2/1(PN)
  Subsystem2/1(TA_com) -> MinMax/1
  MinMax/1 -> Saturation Dynamic/2
  [nA_act] -> Saturation1/1, Subsystem2/2(nA), Saturation2/1, Subsystem1/1(nA_act)
  Lookup Table/1 -> Saturation Dynamic/1
  Lookup Table1/1 -> Saturation Dynamic/3
  Saturation1/1 -> Lookup Table/1
  Saturation2/1 -> Lookup Table1/1
  Subsystem1/1(TA_com) -> MinMax/2
  Saturation Dynamic/1 -> TA_com/1

== system EMT/Control Unit/Control/Prepare Stage/motorB torque/Subsystem1 ==
  nB_act : Inport
  Constant1 : Constant  Value=min(TB_min_map)
  Constant2 : Constant  Value=max(TB_max_map)
  Memory2 : Memory
  Switch2 : Switch  Criteria=u2 > Threshold  SaturateOnIntegerOverflow=off  InputSameDT=off
  TB_com : Outport
  wires:
  Memory2/1 -> Switch2/2
  Switch2/1 -> TB_com/1
  Constant1/1 -> Switch2/1
  Constant2/1 -> Switch2/3
  nB_act/1 -> Memory2/1

== system EMT/Control Unit/Control/Prepare Stage/motorZ torque/Subsystem1 ==
  nZ_act : Inport
  Constant3 : Constant  Value=0
  Memory5 : Memory
  PID Controller2 : simulink_need_slupdate/PID Controller  P=2  I=0.01  D=0.1
  Sum1 : Sum  Inputs=+-
  TZ_com : Outport
  wires:
  Memory5/1 -> Sum1/2
  Constant3/1 -> Sum1/1
  nZ_act/1 -> Memory5/1
  Sum1/1 -> PID Controller2/1
  PID Controller2/1 -> TZ_com/1

== system EMT/Control Unit/Control/Shift Stage/EVT1->EVT2/brack force ==
  Fb_com : Outport
  wires:
  [Fb_ref] -> Fb_com/1

== system EMT/Control Unit/Control/Shift Stage/EVT1->EVT2/clutches condition ==
  note: Z2
  Compare To Constant2 : simulink/Logic and Bit Operations/Compare To Constant  relop=<=  const=0.6  OutDataTypeStr=uint8
  Constant1 : Constant
  Constant2 : Constant  Value=0
  Constant4 : Constant
  Data Type Conversion : DataTypeConversion  SaturateOnIntegerOverflow=off  RndMeth=Floor
  Memory2 : Memory
  Mux1 : Mux
  clutch_com : Outport
  wires:
  Data Type Conversion/1 -> Mux1/3
  Memory2/1 -> Compare To Constant2/1
  [Press_C1] -> Memory2/1
  Constant4/1 -> Mux1/4  "C1"
  Compare To Constant2/1 -> Data Type Conversion/1
  Constant2/1 -> Mux1/2  "Z1"
  Constant1/1 -> Mux1/1  "C0"
  Mux1/1 -> clutch_com/1

== system EMT/Control Unit/Control/Shift Stage/EVT1->EVT2/engine swich ==
  Constant1 : Constant
  engine_swich : Outport
  wires:
  Constant1/1 -> engine_swich/1

== system EMT/Control Unit/Control/Shift Stage/EVT1->EVT2/engine torque ==
  Te_com : Outport
  wires:
  [Te_ref] -> Te_com/1

== system EMT/Control Unit/Control/Shift Stage/EVT1->EVT2/motorA torque ==
  TA_com : Outport
  wires:
  [TA_ref] -> TA_com/1

== system EMT/Control Unit/Control/Shift Stage/EVT1->EVT2/motorB torque ==
  TB_com : Outport
  wires:
  [TB_ref] -> TB_com/1

== system EMT/Control Unit/Control/Shift Stage/EVT1->EVT2/motorZ torque ==
  TZ_com : Outport
  wires:
  [TZ_ref] -> TZ_com/1

== system EMT/Control Unit/Control/Shift Stage/EVT2->EVT1/brack force ==
  Fb_com : Outport
  wires:
  [Fb_ref] -> Fb_com/1

== system EMT/Control Unit/Control/Shift Stage/EVT2->EVT1/clutches condition ==
  note: C1
  Compare To Constant2 : simulink/Logic and Bit Operations/Compare To Constant  relop=<=  const=0.6  OutDataTypeStr=uint8
  Constant1 : Constant
  Constant2 : Constant  Value=0
  Constant3 : Constant
  Data Type Conversion : DataTypeConversion  SaturateOnIntegerOverflow=off  RndMeth=Floor
  Memory2 : Memory
  Mux1 : Mux
  clutch_com : Outport
  wires:
  Data Type Conversion/1 -> Mux1/4
  Memory2/1 -> Compare To Constant2/1
  [Press_Z2] -> Memory2/1
  Compare To Constant2/1 -> Data Type Conversion/1
  Constant3/1 -> Mux1/3  "Z2"
  Constant2/1 -> Mux1/2  "Z1"
  Constant1/1 -> Mux1/1  "C0"
  Mux1/1 -> clutch_com/1

== system EMT/Control Unit/Control/Shift Stage/EVT2->EVT1/engine swich ==
  Constant1 : Constant
  engine_swich : Outport
  wires:
  Constant1/1 -> engine_swich/1

== system EMT/Control Unit/Control/Shift Stage/EVT2->EVT1/engine torque ==
  Te_com : Outport
  wires:
  [Te_ref] -> Te_com/1

== system EMT/Control Unit/Control/Shift Stage/EVT2->EVT1/motorA torque ==
  TA_com : Outport
  wires:
  [TA_ref] -> TA_com/1

== system EMT/Control Unit/Control/Shift Stage/EVT2->EVT1/motorB torque ==
  TB_com : Outport
  wires:
  [TB_ref] -> TB_com/1

== system EMT/Control Unit/Control/Shift Stage/EVT2->EVT1/motorZ torque ==
  Lookup Table : Lookup  InputValues=nZ_map  Table=TZ_max_map  SaturateOnIntegerOverflow=off
  Lookup Table1 : Lookup  InputValues=nZ_map  Table=TZ_min_map  SaturateOnIntegerOverflow=off
  Saturation Dynamic : simulink/Discontinuities/Saturation Dynamic  OutMin=[]  OutMax=[]  OutDataTypeStr=Inherit: Same as second input  OutDataType=sfix(16)  OutScaling=2^-10  DoSatur=off
  Saturation1 : Saturate  UpperLimit=max(nZ_map)  LowerLimit=min(nZ_map)
  Saturation2 : Saturate  UpperLimit=max(nZ_map)  LowerLimit=min(nZ_map)
  Subsystem1 : Subsystem
  TZ_com : Outport
  wires:
  Saturation Dynamic/1 -> TZ_com/1
  [nZ_act] -> Saturation1/1, Saturation2/1, Subsystem1/1(nZ_act)
  Lookup Table/1 -> Saturation Dynamic/1
  Lookup Table1/1 -> Saturation Dynamic/3
  Saturation1/1 -> Lookup Table/1
  Saturation2/1 -> Lookup Table1/1
  Subsystem1/1(TZ_com) -> Saturation Dynamic/2

== system EMT/Control Unit/Driver/Electric Power Requirement/Subsystem4/Subsystem4 ==
  11 : Constant
  21 : Constant  Value=2
  22 : Constant  Value=3
  31 : Constant  Value=4
  0.1 : Outport
  0.01 : Outport  Port=2
  10 : Outport  Port=3
  100 : Outport  Port=4
  wires:
  31/1 -> 100/1
  22/1 -> 10/1
  21/1 -> 0.01/1
  11/1 -> 0.1/1

== system EMT/Control Unit/Driver/Electric Power Requirement/Subsystem4/Subsystem6 ==
  11 : Constant
  21 : Constant  Value=2
  22 : Constant  Value=3
  31 : Constant  Value=4
  1 : Outport
  2 : Outport  Port=2
  3 : Outport  Port=3
  4 : Outport  Port=4
  wires:
  11/1 -> 1/1
  21/1 -> 2/1
  22/1 -> 3/1
  31/1 -> 4/1

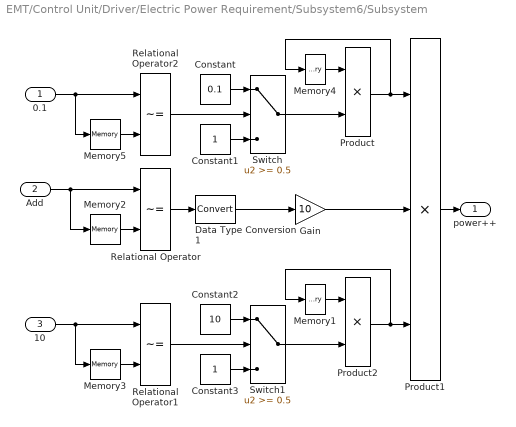
== system EMT/Control Unit/Driver/Electric Power Requirement/Subsystem6/Subsystem ==
  0.1 : Inport
  Add : Inport  Port=2
  10 : Inport  Port=3
  Constant : Constant  Value=0.1
  Constant1 : Constant
  Constant2 : Constant  Value=10
  Constant3 : Constant
  Data Type Conversion1 : DataTypeConversion  SaturateOnIntegerOverflow=off  RndMeth=Floor
  Gain : Gain  Gain=10
  Memory1 : Memory  InitialCondition=1
  Memory2 : Memory
  Memory3 : Memory
  Memory4 : Memory  InitialCondition=1
  Memory5 : Memory
  Product : Product  RndMeth=Zero
  Product1 : Product  Inputs=3  RndMeth=Zero
  Product2 : Product  RndMeth=Zero
  Relational Operator : RelationalOperator  Operator=~=  OutDataTypeStr=boolean  InputSameDT=off
  Relational Operator1 : RelationalOperator  Operator=~=  OutDataTypeStr=boolean  InputSameDT=off
  Relational Operator2 : RelationalOperator  Operator=~=  OutDataTypeStr=boolean  InputSameDT=off
  Switch : Switch  Threshold=0.5  SaturateOnIntegerOverflow=off  InputSameDT=off
  Switch1 : Switch  Threshold=0.5  SaturateOnIntegerOverflow=off  InputSameDT=off
  power++ : Outport
  wires:
  Memory2/1 -> Relational Operator/2
  Add/1 -> Relational Operator/1, Memory2/1
  Relational Operator/1 -> Data Type Conversion1/1
  Data Type Conversion1/1 -> Gain/1
  Product/1 -> Memory4/1, Product1/1
  Memory4/1 -> Product/1
  Memory5/1 -> Relational Operator2/2
  Relational Operator2/1 -> Switch/2
  0.1/1 -> Memory5/1, Relational Operator2/1
  Constant/1 -> Switch/1
  Constant1/1 -> Switch/3
  Switch/1 -> Product/2
  Product1/1 -> power++/1
  Product2/1 -> Memory1/1, Product1/3
  Memory1/1 -> Product2/1
  Memory3/1 -> Relational Operator1/2
  Relational Operator1/1 -> Switch1/2
  10/1 -> Relational Operator1/1, Memory3/1
  Constant2/1 -> Switch1/1
  Constant3/1 -> Switch1/3
  Switch1/1 -> Product2/2
  Gain/1 -> Product1/2

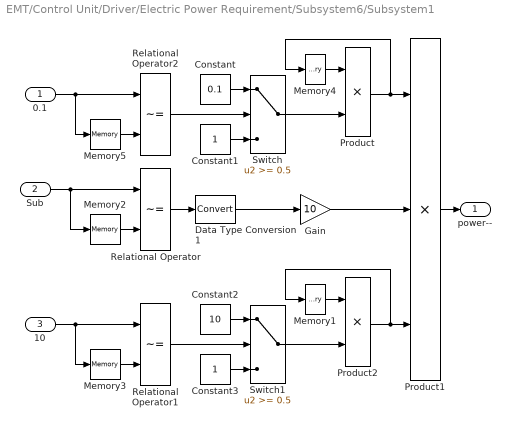
== system EMT/Control Unit/Driver/Electric Power Requirement/Subsystem6/Subsystem1 ==
  0.1 : Inport
  Sub : Inport  Port=2
  10 : Inport  Port=3
  Constant : Constant  Value=0.1
  Constant1 : Constant
  Constant2 : Constant  Value=10
  Constant3 : Constant
  Data Type Conversion1 : DataTypeConversion  SaturateOnIntegerOverflow=off  RndMeth=Floor
  Gain : Gain  Gain=10
  Memory1 : Memory  InitialCondition=1
  Memory2 : Memory
  Memory3 : Memory
  Memory4 : Memory  InitialCondition=1
  Memory5 : Memory
  Product : Product  RndMeth=Zero
  Product1 : Product  Inputs=3  RndMeth=Zero
  Product2 : Product  RndMeth=Zero
  Relational Operator : RelationalOperator  Operator=~=  OutDataTypeStr=boolean  InputSameDT=off
  Relational Operator1 : RelationalOperator  Operator=~=  OutDataTypeStr=boolean  InputSameDT=off
  Relational Operator2 : RelationalOperator  Operator=~=  OutDataTypeStr=boolean  InputSameDT=off
  Switch : Switch  Threshold=0.5  SaturateOnIntegerOverflow=off  InputSameDT=off
  Switch1 : Switch  Threshold=0.5  SaturateOnIntegerOverflow=off  InputSameDT=off
  power-- : Outport
  wires:
  Switch1/1 -> Product2/2
  Constant3/1 -> Switch1/3
  Constant2/1 -> Switch1/1
  10/1 -> Memory3/1, Relational Operator1/1
  Relational Operator1/1 -> Switch1/2
  Memory3/1 -> Relational Operator1/2
  Memory1/1 -> Product2/1
  Product2/1 -> Product1/3, Memory1/1
  Product1/1 -> power--/1
  Switch/1 -> Product/2
  Constant1/1 -> Switch/3
  Constant/1 -> Switch/1
  0.1/1 -> Relational Operator2/1, Memory5/1
  Relational Operator2/1 -> Switch/2
  Memory5/1 -> Relational Operator2/2
  Memory4/1 -> Product/1
  Product/1 -> Product1/1, Memory4/1
  Data Type Conversion1/1 -> Gain/1
  Relational Operator/1 -> Data Type Conversion1/1
  Sub/1 -> Memory2/1, Relational Operator/1
  Memory2/1 -> Relational Operator/2
  Gain/1 -> Product1/2

== system EMT/Control Unit/Driver/Grade Angle/Subsystem4/Subsystem4 ==
  11 : Constant
  21 : Constant  Value=2
  22 : Constant  Value=3
  31 : Constant  Value=4
  0.1 : Outport
  0.01 : Outport  Port=2
  10 : Outport  Port=3
  100 : Outport  Port=4
  wires:
  31/1 -> 100/1
  22/1 -> 10/1
  21/1 -> 0.01/1
  11/1 -> 0.1/1

== system EMT/Control Unit/Driver/Grade Angle/Subsystem4/Subsystem6 ==
  11 : Constant
  21 : Constant  Value=2
  22 : Constant  Value=3
  31 : Constant  Value=4
  1 : Outport
  2 : Outport  Port=2
  3 : Outport  Port=3
  4 : Outport  Port=4
  wires:
  11/1 -> 1/1
  21/1 -> 2/1
  22/1 -> 3/1
  31/1 -> 4/1

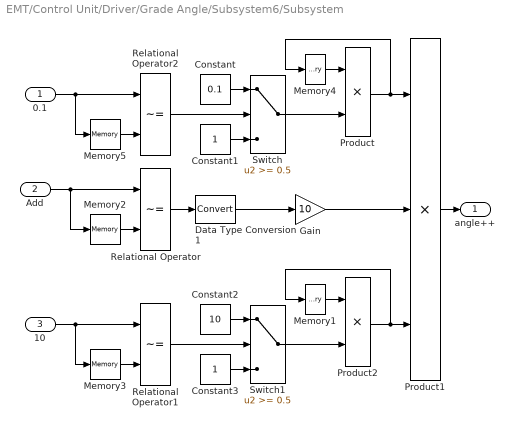
== system EMT/Control Unit/Driver/Grade Angle/Subsystem6/Subsystem ==
  0.1 : Inport
  Add : Inport  Port=2
  10 : Inport  Port=3
  Constant : Constant  Value=0.1
  Constant1 : Constant
  Constant2 : Constant  Value=10
  Constant3 : Constant
  Data Type Conversion1 : DataTypeConversion  SaturateOnIntegerOverflow=off  RndMeth=Floor
  Gain : Gain  Gain=10
  Memory1 : Memory  InitialCondition=1
  Memory2 : Memory
  Memory3 : Memory
  Memory4 : Memory  InitialCondition=1
  Memory5 : Memory
  Product : Product  RndMeth=Zero
  Product1 : Product  Inputs=3  RndMeth=Zero
  Product2 : Product  RndMeth=Zero
  Relational Operator : RelationalOperator  Operator=~=  OutDataTypeStr=boolean  InputSameDT=off
  Relational Operator1 : RelationalOperator  Operator=~=  OutDataTypeStr=boolean  InputSameDT=off
  Relational Operator2 : RelationalOperator  Operator=~=  OutDataTypeStr=boolean  InputSameDT=off
  Switch : Switch  Threshold=0.5  SaturateOnIntegerOverflow=off  InputSameDT=off
  Switch1 : Switch  Threshold=0.5  SaturateOnIntegerOverflow=off  InputSameDT=off
  angle++ : Outport
  wires:
  Memory2/1 -> Relational Operator/2
  Add/1 -> Relational Operator/1, Memory2/1
  Relational Operator/1 -> Data Type Conversion1/1
  Data Type Conversion1/1 -> Gain/1
  Product/1 -> Memory4/1, Product1/1
  Memory4/1 -> Product/1
  Memory5/1 -> Relational Operator2/2
  Relational Operator2/1 -> Switch/2
  0.1/1 -> Memory5/1, Relational Operator2/1
  Constant/1 -> Switch/1
  Constant1/1 -> Switch/3
  Switch/1 -> Product/2
  Product1/1 -> angle++/1
  Product2/1 -> Memory1/1, Product1/3
  Memory1/1 -> Product2/1
  Memory3/1 -> Relational Operator1/2
  Relational Operator1/1 -> Switch1/2
  10/1 -> Relational Operator1/1, Memory3/1
  Constant2/1 -> Switch1/1
  Constant3/1 -> Switch1/3
  Switch1/1 -> Product2/2
  Gain/1 -> Product1/2
